simulink model "industrial_dc_motor_drive_architecture"  (R2024b)
settings: Solver=VariableStepAuto  StartTime=0.0  StopTime=10.0  RelTol=1e-3
settings Model: Creator=Taha  LastModifiedBy=Taha

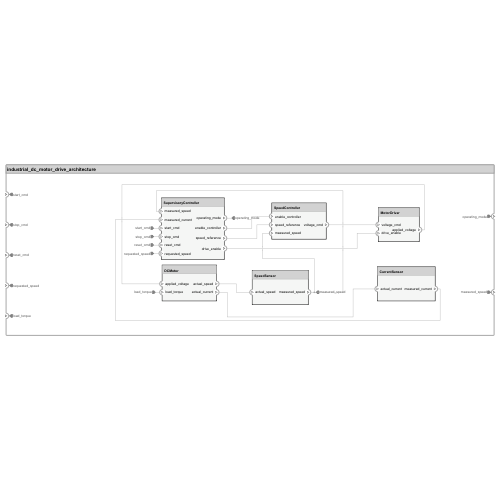
[thumbnail: Simulink's stored preview of the top-level diagram]
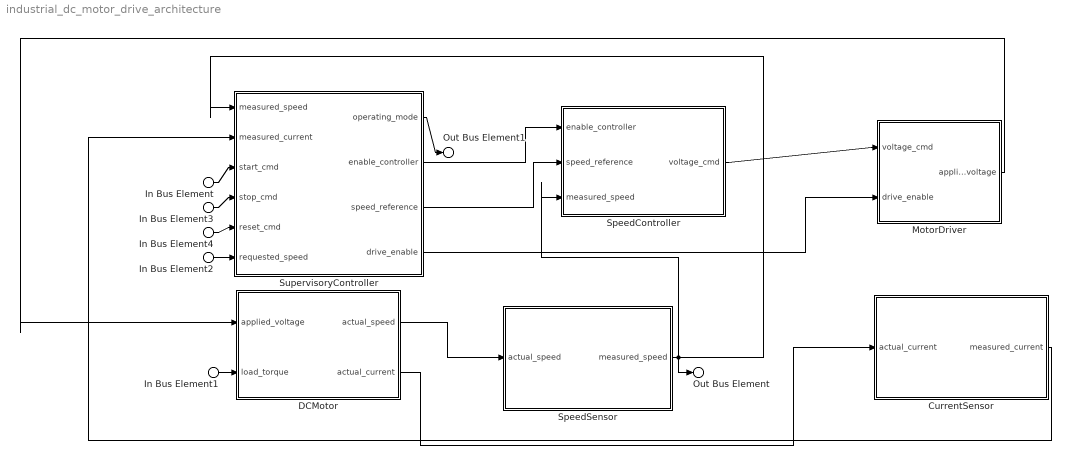
== system industrial_dc_motor_drive_architecture ==
  In Bus Element : Inport  PortName=start_cmd
  In Bus Element3 : Inport  Port=2  PortName=stop_cmd
  In Bus Element4 : Inport  Port=3  PortName=reset_cmd
  In Bus Element2 : Inport  Port=4  PortName=requested_speed
  In Bus Element1 : Inport  Port=5  PortName=load_torque
  CurrentSensor : Subsystem
      settings: PortSchema="{\"entries\":[{\"content\":{\"headerSize\":26,\"margin\":15,\"minimumSpacing\":25,\"sides\":[{\"content\":{\"connectorIds\":[\"In1\"]},\"type\":\"ConnectorPlacement.EquallySpacedRectSide\",\"uuid\":\"dbd382b1-e713-4160-adb1-be9b055fe265\"},{\"content\":{\"connectorIds\":[\"Out1\"],\"side\":\"RIGHT\"},\"type\":\"ConnectorPlacement.EquallySpacedRectSide\",\"uuid\":\"b73b0145-1049-415b-a22b-629b5ccbecc8\"},{\"content\":{\"side\":\"TOP\"},\"type\":\"ConnectorPlacement.EquallySpacedRectSide\",\"uuid\":\"172f227d-2ad9-4c5c-9133-1f107f696cf3\"}]},\"type\":\"ConnectorPlacement.EquallySpacedConnector\",\"uuid\":\"58c77bf4-ebe2-44bc-b7d3-ea25b18aa574\"}],\"packageUris\":[\"http://schema.mathworks.com/mf0/Connector/R2020b\"],\"version\":\"1.0\"}"
  DCMotor : Subsystem
      settings: PortSchema="{\"entries\":[{\"content\":{\"headerSize\":26,\"margin\":15,\"minimumSpacing\":25,\"sides\":[{\"content\":{\"connectorIds\":[\"In1\",\"In2\"]},\"type\":\"ConnectorPlacement.EquallySpacedRectSide\",\"uuid\":\"dbd382b1-e713-4160-adb1-be9b055fe265\"},{\"content\":{\"connectorIds\":[\"Out1\",\"Out2\"],\"side\":\"RIGHT\"},\"type\":\"ConnectorPlacement.EquallySpacedRectSide\",\"uuid\":\"b73b0145-1049-415b-a22b-629b5ccbecc8\"},{\"content\":{\"side\":\"TOP\"},\"type\":\"ConnectorPlacement.EquallySpacedRectSide\",\"uuid\":\"172f227d-2ad9-4c5c-9133-1f107f696cf3\"}]},\"type\":\"ConnectorPlacement.EquallySpacedConnector\",\"uuid\":\"58c77bf4-ebe2-44bc-b7d3-ea25b18aa574\"}],\"packageUris\":[\"http://schema.mathworks.com/mf0/Connector/R2020b\"],\"version\":\"1.0\"}"
  MotorDriver : Subsystem
      settings: PortSchema="{\"entries\":[{\"content\":{\"headerSize\":26,\"margin\":15,\"minimumSpacing\":25,\"sides\":[{\"content\":{\"connectorIds\":[\"In1\",\"In2\"]},\"type\":\"ConnectorPlacement.EquallySpacedRectSide\",\"uuid\":\"dbd382b1-e713-4160-adb1-be9b055fe265\"},{\"content\":{\"connectorIds\":[\"Out1\"],\"side\":\"RIGHT\"},\"type\":\"ConnectorPlacement.EquallySpacedRectSide\",\"uuid\":\"b73b0145-1049-415b-a22b-629b5ccbecc8\"},{\"content\":{\"side\":\"TOP\"},\"type\":\"ConnectorPlacement.EquallySpacedRectSide\",\"uuid\":\"172f227d-2ad9-4c5c-9133-1f107f696cf3\"}]},\"type\":\"ConnectorPlacement.EquallySpacedConnector\",\"uuid\":\"58c77bf4-ebe2-44bc-b7d3-ea25b18aa574\"}],\"packageUris\":[\"http://schema.mathworks.com/mf0/Connector/R2020b\"],\"version\":\"1.0\"}"
  SpeedController : Subsystem
      settings: PortSchema="{\"entries\":[{\"content\":{\"headerSize\":26,\"margin\":15,\"minimumSpacing\":25,\"sides\":[{\"content\":{\"connectorIds\":[\"In1\",\"In2\",\"In3\"]},\"type\":\"ConnectorPlacement.EquallySpacedRectSide\",\"uuid\":\"dbd382b1-e713-4160-adb1-be9b055fe265\"},{\"content\":{\"connectorIds\":[\"Out1\"],\"side\":\"RIGHT\"},\"type\":\"ConnectorPlacement.EquallySpacedRectSide\",\"uuid\":\"b73b0145-1049-415b-a22b-629b5ccbecc8\"},{\"content\":{\"side\":\"TOP\"},\"type\":\"ConnectorPlacement.EquallySpacedRectSide\",\"uuid\":\"172f227d-2ad9-4c5c-9133-1f107f696cf3\"}]},\"type\":\"ConnectorPlacement.EquallySpacedConnector\",\"uuid\":\"58c77bf4-ebe2-44bc-b7d3-ea25b18aa574\"}],\"packageUris\":[\"http://schema.mathworks.com/mf0/Connector/R2020b\"],\"version\":\"1.0\"}"
  SpeedSensor : Subsystem
      settings: PortSchema="{\"entries\":[{\"content\":{\"headerSize\":26,\"margin\":15,\"minimumSpacing\":25,\"sides\":[{\"content\":{\"connectorIds\":[\"In1\"]},\"type\":\"ConnectorPlacement.EquallySpacedRectSide\",\"uuid\":\"dbd382b1-e713-4160-adb1-be9b055fe265\"},{\"content\":{\"connectorIds\":[\"Out1\"],\"side\":\"RIGHT\"},\"type\":\"ConnectorPlacement.EquallySpacedRectSide\",\"uuid\":\"b73b0145-1049-415b-a22b-629b5ccbecc8\"},{\"content\":{\"side\":\"TOP\"},\"type\":\"ConnectorPlacement.EquallySpacedRectSide\",\"uuid\":\"172f227d-2ad9-4c5c-9133-1f107f696cf3\"}]},\"type\":\"ConnectorPlacement.EquallySpacedConnector\",\"uuid\":\"58c77bf4-ebe2-44bc-b7d3-ea25b18aa574\"}],\"packageUris\":[\"http://schema.mathworks.com/mf0/Connector/R2020b\"],\"version\":\"1.0\"}"
  SupervisoryController : Subsystem
      settings: PortSchema="{\"entries\":[{\"content\":{\"headerSize\":26,\"margin\":15,\"minimumSpacing\":25,\"sides\":[{\"content\":{\"connectorIds\":[\"In1\",\"In2\",\"In3\",\"In4\",\"In5\",\"In6\"]},\"type\":\"ConnectorPlacement.EquallySpacedRectSide\",\"uuid\":\"dbd382b1-e713-4160-adb1-be9b055fe265\"},{\"content\":{\"connectorIds\":[\"Out1\",\"Out2\",\"Out3\",\"Out4\"],\"side\":\"RIGHT\"},\"type\":\"ConnectorPlacement.EquallySpacedRectSide\",\"uuid\":\"b73b0145-1049-415b-a22b-629b5ccbecc8\"},{\"content\":{\"side\":\"TOP\"},\"type\":\"ConnectorPlacement.EquallySpacedRectSide\",\"uuid\":\"172f227d-2ad9-4c5c-9133-1f107f696cf3\"}]},\"type\":\"ConnectorPlacement.EquallySpacedConnector\",\"uuid\":\"58c77bf4-ebe2-44bc-b7d3-ea25b18aa574\"}],\"packageUris\":[\"http://schema.mathworks.com/mf0/Connector/R2020b\"],\"version\":\"1.0\"}"
  Out Bus Element1 : Outport  PortName=operating_mode
  Out Bus Element : Outport  Port=2  PortName=measured_speed
  wires:
  SupervisoryController/2(enable_controller) -> SpeedController/1(enable_controller)
  SupervisoryController/3(speed_reference) -> SpeedController/2(speed_reference)
  SupervisoryController/4(drive_enable) -> MotorDriver/2(drive_enable)
  SpeedController/1(voltage_cmd) -> MotorDriver/1(voltage_cmd)
  MotorDriver/1(applied_voltage) -> DCMotor/1(applied_voltage)
  DCMotor/1(actual_speed) -> SpeedSensor/1(actual_speed)
  DCMotor/2(actual_current) -> CurrentSensor/1(actual_current)
  CurrentSensor/1(measured_current) -> SupervisoryController/2(measured_current)
  SpeedSensor/1(measured_speed) -> SupervisoryController/1(measured_speed), SpeedController/3(measured_speed), Out Bus Element/1
  In Bus Element/1 -> SupervisoryController/3(start_cmd)
  In Bus Element3/1 -> SupervisoryController/4(stop_cmd)
  In Bus Element4/1 -> SupervisoryController/5(reset_cmd)
  In Bus Element2/1 -> SupervisoryController/6(requested_speed)
  In Bus Element1/1 -> DCMotor/2(load_torque)
  SupervisoryController/1(operating_mode) -> Out Bus Element1/1

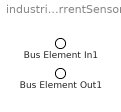
== system industrial_dc_motor_drive_architecture/CurrentSensor ==
  Bus Element In1 : Inport  PortName=actual_current
  Bus Element Out1 : Outport  PortName=measured_current

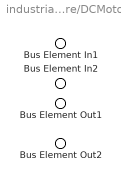
== system industrial_dc_motor_drive_architecture/DCMotor ==
  Bus Element In1 : Inport  PortName=applied_voltage
  Bus Element In2 : Inport  Port=2  PortName=load_torque
  Bus Element Out1 : Outport  PortName=actual_speed
  Bus Element Out2 : Outport  Port=2  PortName=actual_current

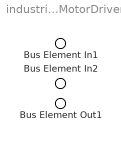
== system industrial_dc_motor_drive_architecture/MotorDriver ==
  Bus Element In1 : Inport  PortName=voltage_cmd
  Bus Element In2 : Inport  Port=2  PortName=drive_enable
  Bus Element Out1 : Outport  PortName=applied_voltage

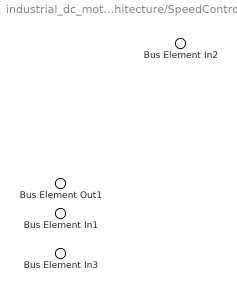
== system industrial_dc_motor_drive_architecture/SpeedController ==
  Bus Element In2 : Inport  PortName=enable_controller
  Bus Element In1 : Inport  Port=2  PortName=speed_reference
  Bus Element In3 : Inport  Port=3  PortName=measured_speed
  Bus Element Out1 : Outport  PortName=voltage_cmd

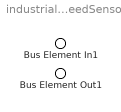
== system industrial_dc_motor_drive_architecture/SpeedSensor ==
  Bus Element In1 : Inport  PortName=actual_speed
  Bus Element Out1 : Outport  PortName=measured_speed

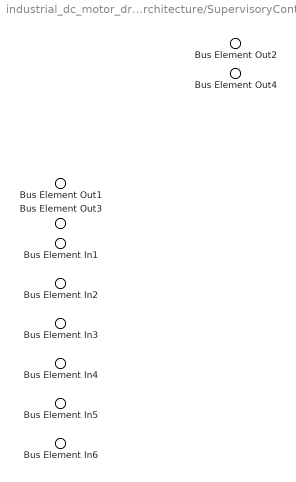
== system industrial_dc_motor_drive_architecture/SupervisoryController ==
  Bus Element In1 : Inport  PortName=measured_speed
  Bus Element In2 : Inport  Port=2  PortName=measured_current
  Bus Element In3 : Inport  Port=3  PortName=start_cmd
  Bus Element In4 : Inport  Port=4  PortName=stop_cmd
  Bus Element In5 : Inport  Port=5  PortName=reset_cmd
  Bus Element In6 : Inport  Port=6  PortName=requested_speed
  Bus Element Out4 : Outport  PortName=operating_mode
  Bus Element Out2 : Outport  Port=2  PortName=enable_controller
  Bus Element Out1 : Outport  Port=3  PortName=speed_reference
  Bus Element Out3 : Outport  Port=4  PortName=drive_enable
